simulink model "dc_motor"  (R2024b)
settings: Solver=VariableStepAuto  StartTime=0.0  StopTime=60  RelTol=1e-3
InitFcn:
  | R = 5.5
  | L = 0.028
  | J = 0.5
  | k = 1
  | kp = 5.684847145
  | ki = 1.7247
  | phi = 0.5
libraries: slpidlib x2, simulink x1, spsTriangleGeneratorLib x1
settings Model: Creator=rohan  LastModifiedBy=rohan

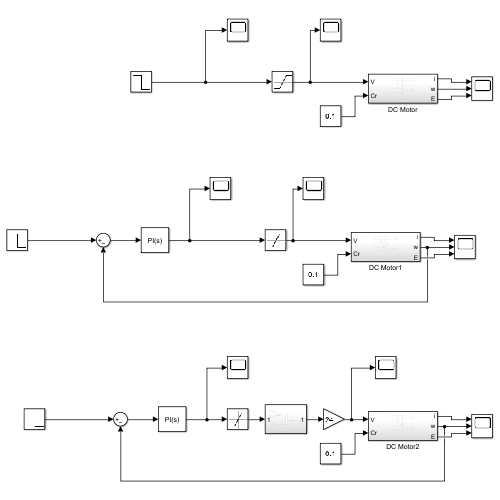
[thumbnail: Simulink's stored preview of the top-level diagram]
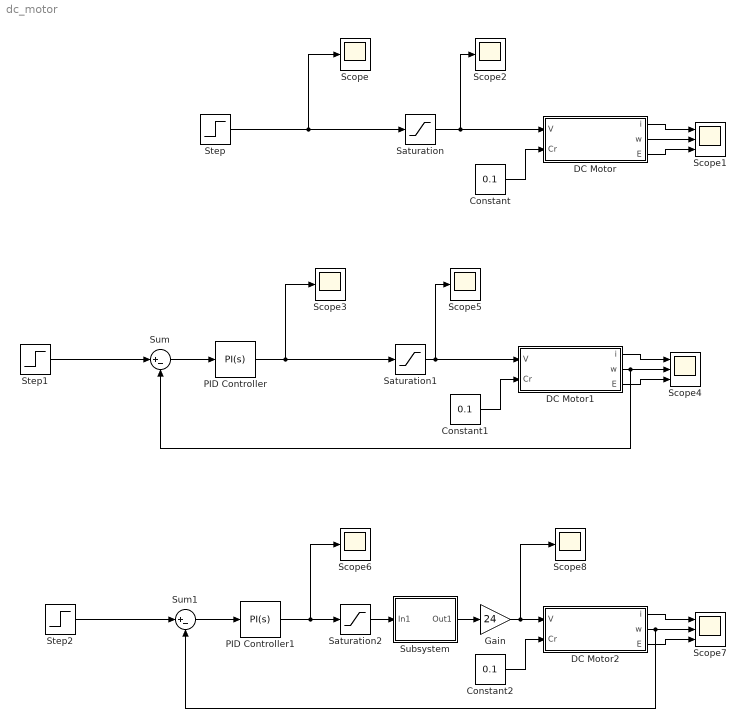
== system dc_motor ==
  Constant : Constant  Value=0.1
  Constant1 : Constant  Value=0.1
  Constant2 : Constant  Value=0.1
  DC Motor : Subsystem
  DC Motor1 : Subsystem
  DC Motor2 : Subsystem
  Gain : Gain  Gain=24
  PID Controller : slpidlib/PID Controller  Controller=PI  Form=Parallel  TimeDomain=Continuous-time  UseExternalTs=off  SampleTime=-1  IntegratorMethod=Forward Euler  FilterMethod=Forward Euler  ControllerParametersSource=internal  P=1  I=1  UseKiTs=off  D=0  UseExternalDerivativeSource=off  N=100  UseFilter=on  TunerSelectOption=Transfer Function Based (PID Tuner App)  InitialConditionSource=internal  InitialConditionForIntegrator=0  InitialConditionForFilter=0  DifferentiatorICPrevScaledInput=0  ExternalReset=none  TrackingMode=off  Kt=1  LimitOutput=off  SatLimitsSource=internal  UpperSaturationLimit=inf  LowerSaturationLimit=-inf  LinearizeAsGain=on  AntiWindupMode=none  Kb=1  LimitIntegrator=off  UpperIntegratorSaturationLimit=inf  LowerIntegratorSaturationLimit=-inf  POutMin=[]  POutMax=[]  IOutMin=[]  IOutMax=[]  DOutMin=[]  DOutMax=[]  NOutMin=[]  NOutMax=[]  SumOutMin=[]  SumOutMax=[]  SaturationOutMin=[]  SaturationOutMax=[]  PParamMin=[]  PParamMax=[]  IParamMin=[]  IParamMax=[]  DParamMin=[]  DParamMax=[]  NParamMin=[]  NParamMax=[]  KbParamMin=[]  KbParamMax=[]  KtParamMin=[]  KtParamMax=[]  KbOutMin=[]  KbOutMax=[]  KtOutMin=[]  KtOutMax=[]  IntegratorOutMin=[]  IntegratorOutMax=[]  FilterOutMin=[]  FilterOutMax=[]  SumI1OutMin=[]  SumI1OutMax=[]  SumI2OutMin=[]  SumI2OutMax=[]  SumI3OutMin=[]  SumI3OutMax=[]  SumI4OutMin=[]  SumI4OutMax=[]  SumDOutMin=[]  SumDOutMax=[]  DifferentiatorOutMin=[]  DifferentiatorOutMax=[]  FilterDiffOutCoefMin=[]  FilterDiffOutCoefMax=[]  ReciprocalOutMin=[]  ReciprocalOutMax=[]  SumDenOutMin=[]  SumDenOutMax=[]  SumNumOutMin=[]  SumNumOutMax=[]  DivideOutMin=[]  DivideOutMax=[]  UdiffTsProdOutMin=[]  UdiffTsProdOutMax=[]  NTsProdOutMin=[]  NTsProdOutMax=[]  UintegralTsProdOutMin=[]  UintegralTsProdOutMax=[]  UngainTsProdOutMin=[]  UngainTsProdOutMax=[]  ClampingZeroOutDataTypeStr=Inherit: Inherit via back propagation  ClampingZeroOutMin=[]  ClampingZeroOutMax=[]  FilterDenConstantOutDataTypeStr=Inherit: Inherit via back propagation  FilterDenConstantOutMin=[]  FilterDenConstantOutMax=[]  PCopyOutDataTypeStr=Inherit: Inherit via back propagation  PCopyOutMin=[]  PCopyOutMax=[]  NCopyOutDataTypeStr=Inherit: Inherit via back propagation  NCopyOutMin=[]  NCopyOutMax=[]  IntegratorContinuousStateAttributes=''  IntegratorStateMustResolveToSignalObject=off  IntegratorRTWStateStorageClass=Auto  FilterContinuousStateAttributes=''  FilterStateMustResolveToSignalObject=off  FilterRTWStateStorageClass=Auto  ParallelPVariant=InternalParameters  IdealPVariant=Disabled  IVariant=InternalParameters  DVariant=Disabled  IntegratorVariant=Continuous  SatVariant=Disabled  AWVariant=Passthrough  PCopyVariant=Disabled  TRVariant=Disabled  FdbkBlocksVariant=Forward  IdealPFdbkVariant=Disabled  SatFdbkVariant=Disabled  DerivativeFilterVariant=Disabled  NVariant=Disabled  NCopyVariant=Disabled_SignalSpec  FilterICVariant=Disabled  IntegratorICVariant=InternalICs  ExternalResetVariant=Disabled  TRSumVariant=Passthrough  SumFdbkVariant=Disabled  SumVariant=Sum_PI  TsampFilterVariant=InternalTs  TsampNgainVariant=Passthrough  TsampIntegralVariant=Disabled_SignalSpec  ExternalSaturationOutDataTypeStr=Inherit: Same as second input  DerivativeSourceVariant=Disabled  PreIntVariant=InternalPreInt
  PID Controller1 : slpidlib/PID Controller  Controller=PI  Form=Parallel  TimeDomain=Continuous-time  UseExternalTs=off  SampleTime=-1  IntegratorMethod=Forward Euler  FilterMethod=Forward Euler  ControllerParametersSource=internal  P=kp  I=ki  UseKiTs=off  D=0  UseExternalDerivativeSource=off  N=100  UseFilter=on  TunerSelectOption=Transfer Function Based (PID Tuner App)  InitialConditionSource=internal  InitialConditionForIntegrator=0  InitialConditionForFilter=0  DifferentiatorICPrevScaledInput=0  ExternalReset=none  TrackingMode=off  Kt=1  LimitOutput=off  SatLimitsSource=internal  UpperSaturationLimit=inf  LowerSaturationLimit=-inf  LinearizeAsGain=on  AntiWindupMode=none  Kb=1  LimitIntegrator=off  UpperIntegratorSaturationLimit=inf  LowerIntegratorSaturationLimit=-inf  POutMin=[]  POutMax=[]  IOutMin=[]  IOutMax=[]  DOutMin=[]  DOutMax=[]  NOutMin=[]  NOutMax=[]  SumOutMin=[]  SumOutMax=[]  SaturationOutMin=[]  SaturationOutMax=[]  PParamMin=[]  PParamMax=[]  IParamMin=[]  IParamMax=[]  DParamMin=[]  DParamMax=[]  NParamMin=[]  NParamMax=[]  KbParamMin=[]  KbParamMax=[]  KtParamMin=[]  KtParamMax=[]  KbOutMin=[]  KbOutMax=[]  KtOutMin=[]  KtOutMax=[]  IntegratorOutMin=[]  IntegratorOutMax=[]  FilterOutMin=[]  FilterOutMax=[]  SumI1OutMin=[]  SumI1OutMax=[]  SumI2OutMin=[]  SumI2OutMax=[]  SumI3OutMin=[]  SumI3OutMax=[]  SumI4OutMin=[]  SumI4OutMax=[]  SumDOutMin=[]  SumDOutMax=[]  DifferentiatorOutMin=[]  DifferentiatorOutMax=[]  FilterDiffOutCoefMin=[]  FilterDiffOutCoefMax=[]  ReciprocalOutMin=[]  ReciprocalOutMax=[]  SumDenOutMin=[]  SumDenOutMax=[]  SumNumOutMin=[]  SumNumOutMax=[]  DivideOutMin=[]  DivideOutMax=[]  UdiffTsProdOutMin=[]  UdiffTsProdOutMax=[]  NTsProdOutMin=[]  NTsProdOutMax=[]  UintegralTsProdOutMin=[]  UintegralTsProdOutMax=[]  UngainTsProdOutMin=[]  UngainTsProdOutMax=[]  ClampingZeroOutDataTypeStr=Inherit: Inherit via back propagation  ClampingZeroOutMin=[]  ClampingZeroOutMax=[]  FilterDenConstantOutDataTypeStr=Inherit: Inherit via back propagation  FilterDenConstantOutMin=[]  FilterDenConstantOutMax=[]  PCopyOutDataTypeStr=Inherit: Inherit via back propagation  PCopyOutMin=[]  PCopyOutMax=[]  NCopyOutDataTypeStr=Inherit: Inherit via back propagation  NCopyOutMin=[]  NCopyOutMax=[]  IntegratorContinuousStateAttributes=''  IntegratorStateMustResolveToSignalObject=off  IntegratorRTWStateStorageClass=Auto  FilterContinuousStateAttributes=''  FilterStateMustResolveToSignalObject=off  FilterRTWStateStorageClass=Auto  ParallelPVariant=InternalParameters  IdealPVariant=Disabled  IVariant=InternalParameters  DVariant=Disabled  IntegratorVariant=Continuous  SatVariant=Disabled  AWVariant=Passthrough  PCopyVariant=Disabled  TRVariant=Disabled  FdbkBlocksVariant=Forward  IdealPFdbkVariant=Disabled  SatFdbkVariant=Disabled  DerivativeFilterVariant=Disabled  NVariant=Disabled  NCopyVariant=Disabled_SignalSpec  FilterICVariant=Disabled  IntegratorICVariant=InternalICs  ExternalResetVariant=Disabled  TRSumVariant=Passthrough  SumFdbkVariant=Disabled  SumVariant=Sum_PI  TsampFilterVariant=InternalTs  TsampNgainVariant=Passthrough  TsampIntegralVariant=Disabled_SignalSpec  ExternalSaturationOutDataTypeStr=Inherit: Same as second input  DerivativeSourceVariant=Disabled  PreIntVariant=InternalPreInt
  Saturation : Saturate  UpperLimit=24  LowerLimit=0
  Saturation1 : Saturate  UpperLimit=24  LowerLimit=0
  Saturation2 : Saturate  UpperLimit=24  LowerLimit=0
  Scope{,2..3,5..6,8} (6 alike) : Scope
  Scope1 : Scope  NumInputPorts=3
  Scope4 : Scope  NumInputPorts=3
  Scope7 : Scope  NumInputPorts=3
  Step : Step  Time=20  Before=10  After=5  SampleTime=0
  Step1 : Step  Time=20  Before=10  After=5  SampleTime=0
  Step2 : Step  Time=20  Before=10  After=5  SampleTime=0
  Subsystem : Subsystem
  Sum : Sum  Inputs=|+-
  Sum1 : Sum  Inputs=|+-
  wires:
  Step/1 -> Saturation/1, Scope/1
  Constant/1 -> DC Motor/2(Cr)
  DC Motor/1(i) -> Scope1/1
  DC Motor/2(w) -> Scope1/2
  DC Motor/3(E) -> Scope1/3
  Saturation/1 -> Scope2/1, DC Motor/1(V)
  DC Motor1/3(E) -> Scope4/3
  Constant1/1 -> DC Motor1/2(Cr)
  Saturation1/1 -> Scope5/1, DC Motor1/1(V)
  DC Motor1/2(w) -> Scope4/2, Sum/2
  DC Motor1/1(i) -> Scope4/1
  Step1/1 -> Sum/1
  Sum/1 -> PID Controller/1
  PID Controller/1 -> Saturation1/1, Scope3/1
  DC Motor2/1(i) -> Scope7/1
  PID Controller1/1 -> Saturation2/1, Scope6/1
  Constant2/1 -> DC Motor2/2(Cr)
  Saturation2/1 -> Subsystem/1(In1)
  DC Motor2/3(E) -> Scope7/3
  DC Motor2/2(w) -> Scope7/2, Sum1/2
  Step2/1 -> Sum1/1
  Sum1/1 -> PID Controller1/1
  Gain/1 -> Scope8/1, DC Motor2/1(V)
  Subsystem/1(Out1) -> Gain/1

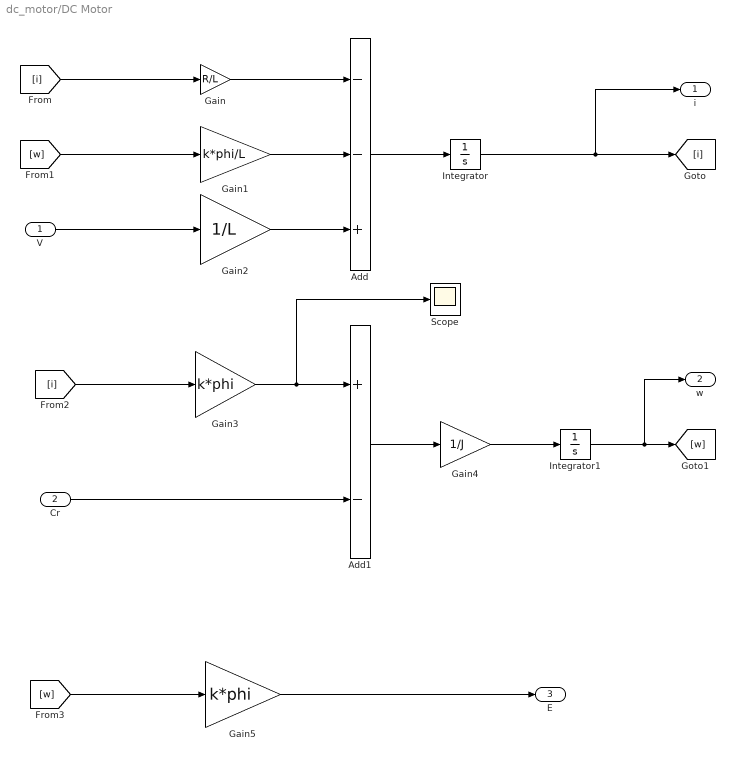
== system dc_motor/DC Motor ==
  V : Inport
  Cr : Inport  Port=2
  Add : Sum  Inputs=--+
  Add1 : Sum  Inputs=+-
  Gain : Gain  Gain=R/L
  Gain1 : Gain  Gain=k*phi/L
  Gain2 : Gain  Gain=1/L
  Gain3 : Gain  Gain=k*phi
  Gain4 : Gain  Gain=1/J
  Gain5 : Gain  Gain=k*phi
  Integrator : Integrator
  Integrator1 : Integrator
  Scope : Scope
  i : Outport
  w : Outport  Port=2
  E : Outport  Port=3
  wires:
  Integrator/1 -> i/1, [i]
  [w] -> Gain5/1
  Gain5/1 -> E/1
  Add1/1 -> Gain4/1
  Gain4/1 -> Integrator1/1
  [i] -> Gain3/1
  Integrator1/1 -> w/1, [w]
  [w] -> Gain1/1
  Gain/1 -> Add/1
  Add/1 -> Integrator/1
  Gain3/1 -> Scope/1, Add1/1
  Cr/1 -> Add1/2
  V/1 -> Gain2/1
  Gain1/1 -> Add/2
  [i] -> Gain/1
  Gain2/1 -> Add/3

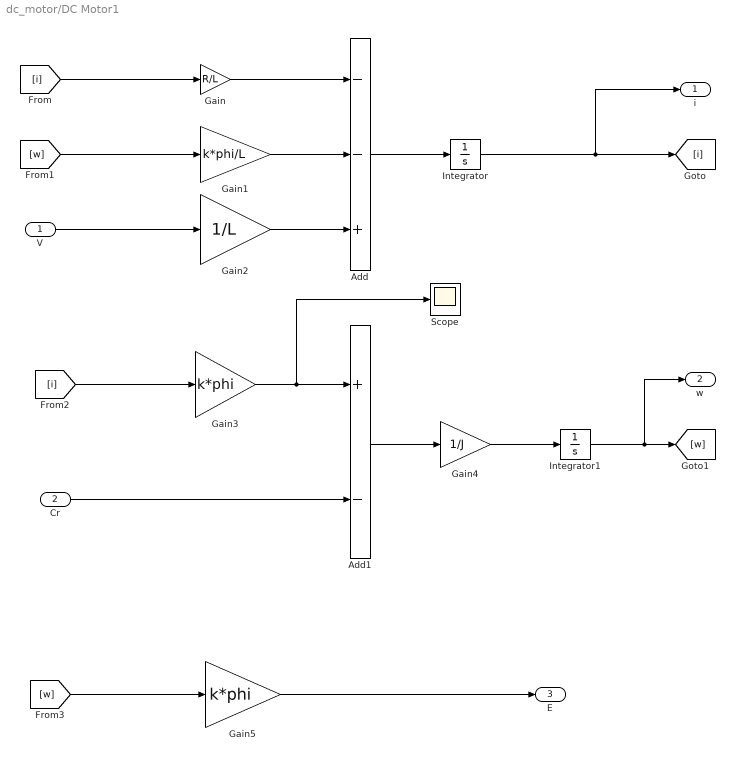
== system dc_motor/DC Motor1 ==
  V : Inport
  Cr : Inport  Port=2
  Add : Sum  Inputs=--+
  Add1 : Sum  Inputs=+-
  Gain : Gain  Gain=R/L
  Gain1 : Gain  Gain=k*phi/L
  Gain2 : Gain  Gain=1/L
  Gain3 : Gain  Gain=k*phi
  Gain4 : Gain  Gain=1/J
  Gain5 : Gain  Gain=k*phi
  Integrator : Integrator
  Integrator1 : Integrator
  Scope : Scope
  i : Outport
  w : Outport  Port=2
  E : Outport  Port=3
  wires:
  Integrator/1 -> i/1, [i]
  [w] -> Gain5/1
  Gain5/1 -> E/1
  Add1/1 -> Gain4/1
  Gain4/1 -> Integrator1/1
  [i] -> Gain3/1
  Integrator1/1 -> w/1, [w]
  [w] -> Gain1/1
  Gain/1 -> Add/1
  Add/1 -> Integrator/1
  Gain3/1 -> Scope/1, Add1/1
  Cr/1 -> Add1/2
  V/1 -> Gain2/1
  Gain1/1 -> Add/2
  [i] -> Gain/1
  Gain2/1 -> Add/3

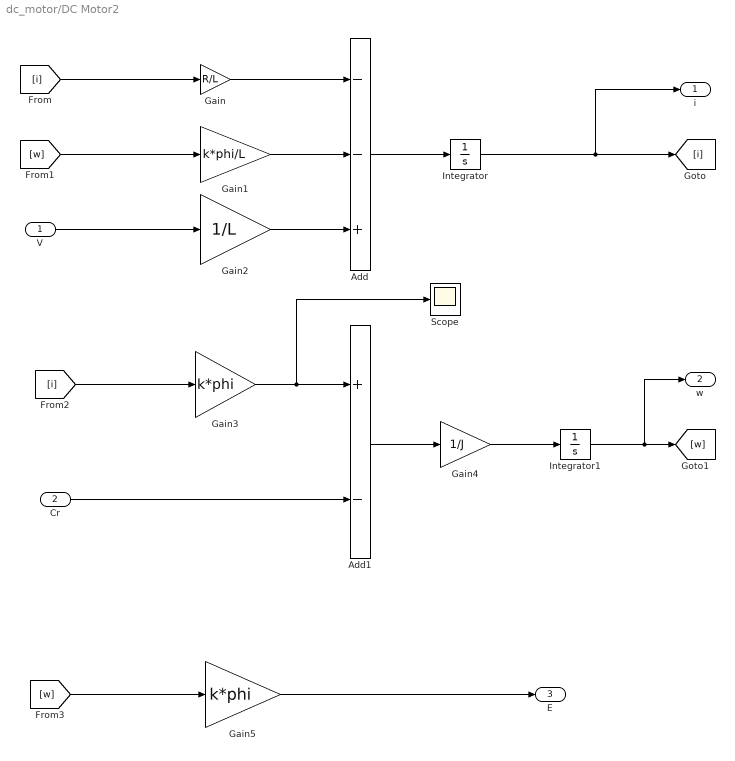
== system dc_motor/DC Motor2 ==
  V : Inport
  Cr : Inport  Port=2
  Add : Sum  Inputs=--+
  Add1 : Sum  Inputs=+-
  Gain : Gain  Gain=R/L
  Gain1 : Gain  Gain=k*phi/L
  Gain2 : Gain  Gain=1/L
  Gain3 : Gain  Gain=k*phi
  Gain4 : Gain  Gain=1/J
  Gain5 : Gain  Gain=k*phi
  Integrator : Integrator
  Integrator1 : Integrator
  Scope : Scope
  i : Outport
  w : Outport  Port=2
  E : Outport  Port=3
  wires:
  Integrator/1 -> i/1, [i]
  [w] -> Gain5/1
  Gain5/1 -> E/1
  Add1/1 -> Gain4/1
  Gain4/1 -> Integrator1/1
  [i] -> Gain3/1
  Integrator1/1 -> w/1, [w]
  [w] -> Gain1/1
  Gain/1 -> Add/1
  Add/1 -> Integrator/1
  Gain3/1 -> Scope/1, Add1/1
  Cr/1 -> Add1/2
  V/1 -> Gain2/1
  Gain1/1 -> Add/2
  [i] -> Gain/1
  Gain2/1 -> Add/3

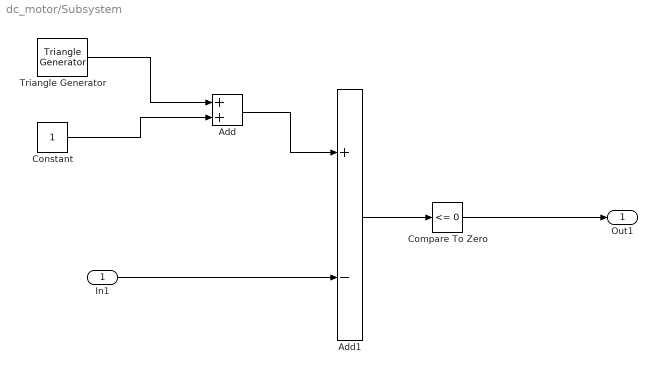
== system dc_motor/Subsystem ==
  In1 : Inport
  Add : Sum
  Add1 : Sum  Inputs=+-
  Compare To Zero : simulink/Logic and Bit Operations/Compare To Zero  relop=<=  OutDataTypeStr=boolean
  Constant : Constant
  Triangle Generator : spsTriangleGeneratorLib/Triangle Generator  Freq=1e3  Phase=90  Ts=0
  Out1 : Outport
  wires:
  Add/1 -> Add1/1
  In1/1 -> Add1/2
  Triangle Generator/1 -> Add/1
  Constant/1 -> Add/2
  Add1/1 -> Compare To Zero/1
  Compare To Zero/1 -> Out1/1
